simulink model "bat4s_check"  (R2025b)
settings: Solver=ode23t  StartTime=0.0  StopTime=10.0  RelTol=1e-3
values from neighbouring files (symbols this model uses):
  bat4s = struct()    [bat4s_params.m]
libraries: bat4s_lib x1, fl_lib x1, nesl_utility x1
settings Model: Creator=SC-Br  LastModifiedBy=SC-Br

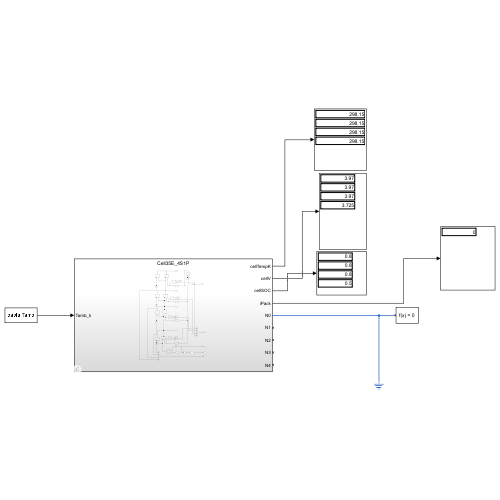
[thumbnail: Simulink's stored preview of the top-level diagram]
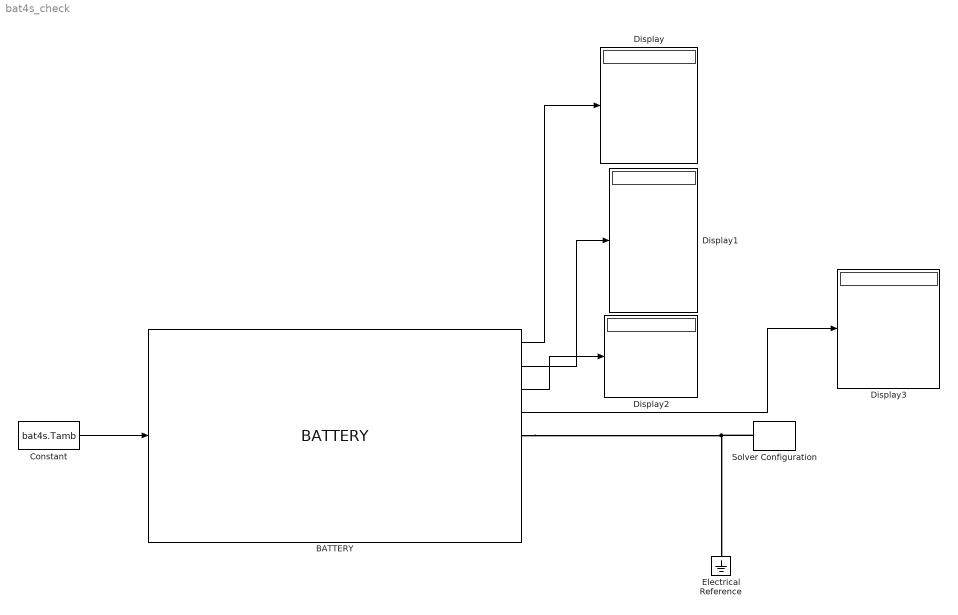
== system bat4s_check ==
  BATTERY : bat4s_lib/BATTERY  SystemSampleTime=-1  VariantActivationTime=update diagram  EmptyChoice=off  PassThrough=off  PassThroughVariantControl=(default)  EmptyChoiceVariantControl=(default)  AllowFlexibleInterface=on  Latency=0  AutoFrameSizeCalculation=off
  Constant : Constant  Value=bat4s.Tamb
  Display{,1..3} (4 alike) : Display
      Display settings: Decimation=2
  Electrical Reference : fl_lib/Electrical/Electrical Elements/Electrical Reference
  Solver Configuration : nesl_utility/Solver Configuration  PhysicalDomain=network_engine_domain  SubClassName=solver  LeftPortType=input  RightPortType=generic  Tones=[]  Harmonics=[]  SimulateNoise=off  Profile=off  UseLocalSampling=off  EnableSwitchedLinearOptims=on  FrequencyDomain=off  UseCCode=off  RelTol=0.001  AbsTol=0.001  MinStep=1e-09  ToWorkspace=off  RevertToSquareIcSolve=off  NumHomotopyIterations=100  PhasorMode=off  PhasorModeNumHarmonics=1  ConsistencySolver=NEWTON_XTOL_AFTER_FTOL  IndexReductionMethod=DerivativeReplacement  DoDC=off  ResidualTolerance=1e-09  ConsistencyTolSource=GLOBAL  ConsistencyAbsTol=0.001  ConsistencyRelTol=0.001  ConsistencyTolFactor=0.001  UseLocalSolver=off  LocalSolverChoice=NE_BACKWARD_EULER_ADVANCER  ResolveIndetEquations=on  FunctionEvalNumThread=1  LocalSolverSampleTime=0.001  DoFixedCost=off  MaxNonlinIter=3  MaxModeIter=2  ComputeImpulses=off  ImpulseIterations=2  LinearAlgebra=auto  LinearAlgebraNumThread=0  EquationFormulation=NE_TIME_EF  DelaysMemoryBudget=1024  AutomaticFiltering=on  FilteringTimeConstant=0.001  PartitionStorageMethod=AS_NEEDED  PartitionMemoryBudget=1024  PartitionMethod=ROBUST  MultibodyUseLocalSolver=off  MultibodyLocalSolverChoice=ODE1  MultibodyLocalSolverSampleTime=0.001
  wires:
  Constant/1 -> BATTERY/1
  BATTERY/1 -> Display/1
  BATTERY/2 -> Display1/1
  BATTERY/3 -> Display2/1
  BATTERY/4 -> Display3/1
  connections:
  BATTERY/RConn1 -- Solver Configuration/RConn1 -- Electrical Reference/LConn1
